simulink model "Problem_2_Celsius_To_Fahrenheit"  (R2026a)
settings: Solver=VariableStepAuto
values from neighbouring files (symbols this model uses):
  X = input(message)    [Problem_2_Celsius_To_Fahrenheit_Run.m]    (also in problem3b.m)
settings Model: Creator=HP  LastModifiedBy=rawad

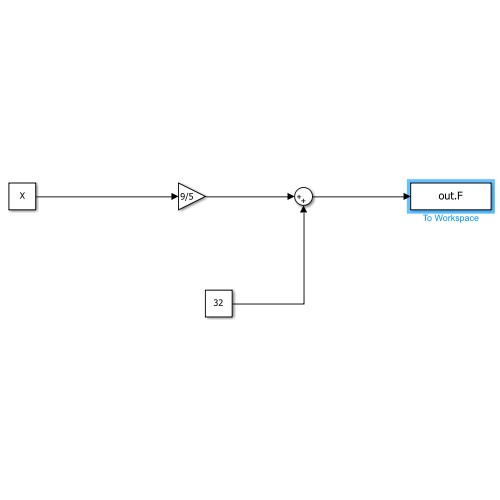
[thumbnail: Simulink's stored preview of the top-level diagram]
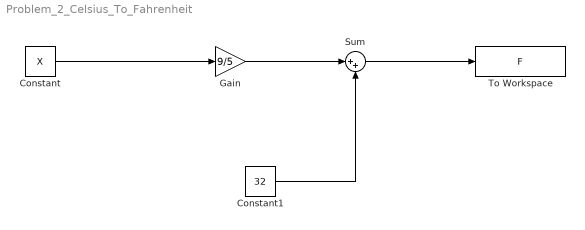
== system Problem_2_Celsius_To_Fahrenheit ==
  Constant : Constant  Value=X
  Constant1 : Constant  Value=32
  Gain : Gain  Gain=9/5
  Sum : Sum  Inputs=|++
  To Workspace : ToWorkspace  VariableName=F  SaveFormat=Timeseries  SampleTime=-1
  wires:
  Constant/1 -> Gain/1
  Gain/1 -> Sum/1
  Constant1/1 -> Sum/2
  Sum/1 -> To Workspace/1
